simulink library "ardupilot_sitl_lib"  (R2018b)
settings: Solver=VariableStepAuto  StartTime=0.0  StopTime=10.0  RelTol=1e-3
libraries: dspnetwork x5, etargetslib x3, $bdroot x2, sensors_lib x2
settings Model: Creator=yannic  LastModifiedBy=yannic

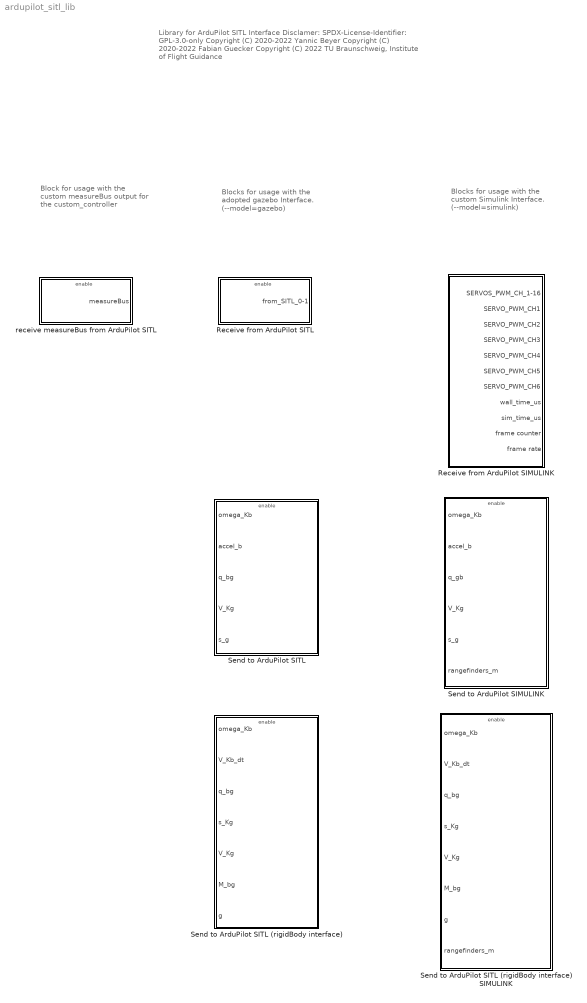
== system ardupilot_sitl_lib ==
  note: Block for usage
      | with the custom
      | measureBus output
      | for the
      | custom_controller
  note: Blocks for usage
      | with the custom
      | Simulink Interface.
      |
      | (--model=simulink)
  note: Blocks for usage
      | with the adopted
      | gazebo Interface.
      |
      | (--model=gazebo)
  note: Library for ArduPilot SITL Interface
      |
      | Disclamer:
      | SPDX-License-Identifier: GPL-3.0-only
      |
      | Copyright (C) 2020-2022 Yannic Beyer
      | Copyright (C) 2020-2022 Fabian Guecker
      | Copyright (C) 2022 TU Braunschweig, Institute of Flight Guidance
  Receive from ArduPilot SIMULINK : Subsystem  mask{IP='127.0.0.1', Port=9002, sample_time=1/400, blocking_time=1}
      mask prompts: sample_time "Sample time"; blocking_time "Blocking time (wait for signal), in s"
  Receive from ArduPilot SITL : Subsystem  mask{idx=[3,1,4,2], IP='127.0.0.1', Port=9002, sample_time=1/400, blocking_time=inf}
      mask prompts: idx "Pick channel indices"; sample_time "Sample time"; blocking_time "Blocking time (wait for signal), in s"
  Send to ArduPilot SIMULINK : Subsystem  mask{IP='127.0.0.1', Port=9003, sample_time=1/400}
      mask prompts: sample_time "Sample time"
      mask DialogControl DescGroupVar Prompt: Send to ArduPilot SITL
      mask DialogControl DescTextVar Prompt: Use rigidBody or sensor data as inputs.
      mask DialogControl Control2 Prompt: The input accel_b is the acceleration measured by an IMU in body frame.
  Send to ArduPilot SITL : Subsystem  mask{IP='127.0.0.1', Port=9003, sample_time=1/400}
      mask prompts: sample_time "Sample time"
      mask DialogControl DescGroupVar Prompt: Send to ArduPilot SITL
      mask DialogControl DescTextVar Prompt: Use rigidBody or sensor data as inputs.
      mask DialogControl Control2 Prompt: The input accel_b is the acceleration measured by an IMU in body frame.
  Send to ArduPilot SITL (rigidBody interface) : Subsystem  mask{IP='127.0.0.1', Port=9003, sample_time=1/400}
      mask prompts: sample_time "Sample time"
      mask DialogControl DescGroupVar Prompt: Send to ArduPilot SITL (rigidBody interface)
      mask DialogControl DescTextVar Prompt: Simply connect rigidBody outputs
  Send to ArduPilot SITL (rigidBody interface) SIMULINK : Subsystem  mask{IP='127.0.0.1', Port=9003, sample_time=1/400}
      mask prompts: sample_time "Sample time"
      mask DialogControl DescGroupVar Prompt: Send to ArduPilot SITL (rigidBody interface)
      mask DialogControl DescTextVar Prompt: Simply connect rigidBody outputs
  receive measureBus from ArduPilot SITL : Subsystem  mask{IP='127.0.0.1', Port=9004, sample_time=1/400, blocking_time=0.001}
      mask prompts: sample_time "Sample time"; blocking_time "Blocking time(wait for signal), in s"
      mask init:
      | num_signals = 40;
      mask DialogControl DescGroupVar Prompt: Receive measureBus from ArduPilot SITL
      mask DialogControl DescTextVar Prompt: This block can be used for debugging of the ArduPilot interface.
      mask DialogControl Control2 Prompt: This block only receives the signals if you uncomment line 3 of mode.h in your ArduPilot fork.

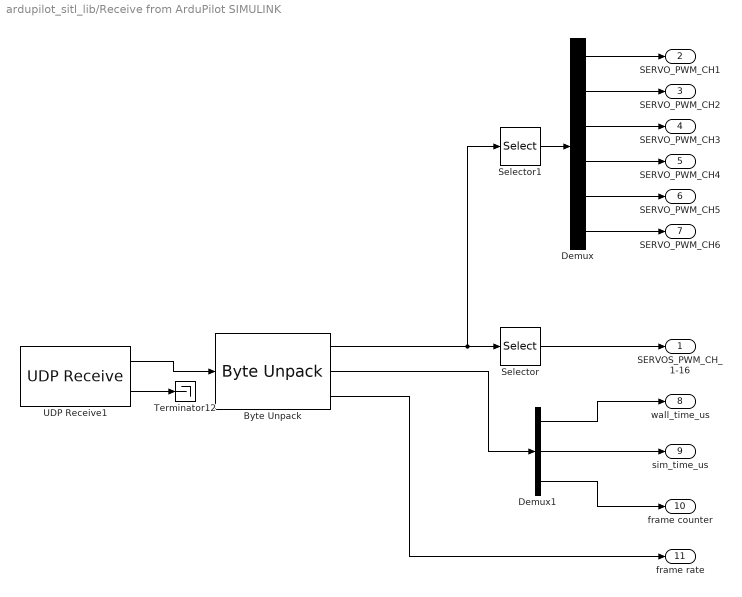
== system ardupilot_sitl_lib/Receive from ArduPilot SIMULINK ==
  Byte Unpack : etargetslib/Byte Unpack  dimensions={[16],[3],[1]}  datatypes={'double','uint32','uint16'}  byteAlign=1
      settings: SourceProductName=/root/.matlab/R2018b/slblocks_master.db is not a database. (file is encrypted or is not a database)
  Demux : Demux  Outputs=6
  Demux1 : Demux  Outputs=3
  Selector : Selector  InputPortWidth=16  IndexOptions=Index vector (dialog)  Indices=[1:16]  OutputSizes=1
  Selector1 : Selector  InputPortWidth=16  IndexOptions=Index vector (dialog)  Indices=[1:6]  OutputSizes=1
  Terminator12 : Terminator
  UDP Receive1 : dspnetwork/UDP Receive  localURL='0.0.0.0'  localPort=Port  remoteURL=IP  remotePort=-1  recvBufferSize=142  dims=142  signalDatatype=uint8  isVarSize=off  showBlockingTime=on  blockingTime=blocking_time  sampletime=sample_time  blockPlatform=HOST
      settings: SourceProductName=DSP System Toolbox  SourceProductBaseCode=DS
  SERVOS_PWM_CH_1-16 : Outport
  SERVO_PWM_CH1 : Outport  Port=2
  SERVO_PWM_CH2 : Outport  Port=3
  SERVO_PWM_CH3 : Outport  Port=4
  SERVO_PWM_CH4 : Outport  Port=5
  SERVO_PWM_CH5 : Outport  Port=6
  SERVO_PWM_CH6 : Outport  Port=7
  wall_time_us : Outport  Port=8
  sim_time_us : Outport  Port=9
  frame counter : Outport  Port=10
  frame rate : Outport  Port=11
  wires:
  UDP Receive1/1 -> Byte Unpack/1
  UDP Receive1/2 -> Terminator12/1
  Selector/1 -> SERVOS_PWM_CH_1-16/1
  Selector1/1 -> Demux/1
  Demux/1 -> SERVO_PWM_CH1/1
  Demux/2 -> SERVO_PWM_CH2/1
  Demux/6 -> SERVO_PWM_CH6/1
  Demux/5 -> SERVO_PWM_CH5/1
  Demux/4 -> SERVO_PWM_CH4/1
  Demux/3 -> SERVO_PWM_CH3/1
  Byte Unpack/2 -> Demux1/1
  Demux1/1 -> wall_time_us/1
  Demux1/2 -> sim_time_us/1
  Byte Unpack/1 -> Selector1/1, Selector/1
  Demux1/3 -> frame counter/1
  Byte Unpack/3 -> frame rate/1

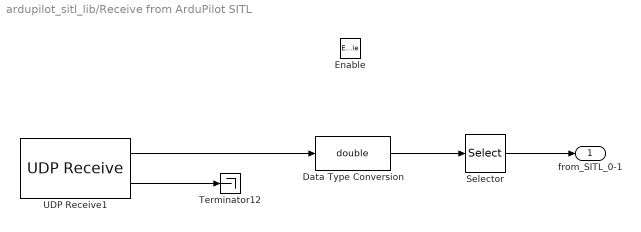
== system ardupilot_sitl_lib/Receive from ArduPilot SITL ==
  Enable : EnablePort
  Data Type Conversion : DataTypeConversion  OutDataTypeStr=double
  Selector : Selector  InputPortWidth=16  IndexOptions=Index vector (dialog)  Indices=idx  OutputSizes=1
  Terminator12 : Terminator
  UDP Receive1 : dspnetwork/UDP Receive  localURL='0.0.0.0'  localPort=Port  remoteURL=IP  remotePort=-1  recvBufferSize=64  dims=16  signalDatatype=single  isVarSize=off  showBlockingTime=on  blockingTime=blocking_time  sampletime=sample_time  blockPlatform=HOST
      settings: SourceProductName=DSP System Toolbox  SourceProductBaseCode=DS
  from_SITL_0-1 : Outport
  wires:
  UDP Receive1/1 -> Data Type Conversion/1
  UDP Receive1/2 -> Terminator12/1
  Data Type Conversion/1 -> Selector/1
  Selector/1 -> from_SITL_0-1/1

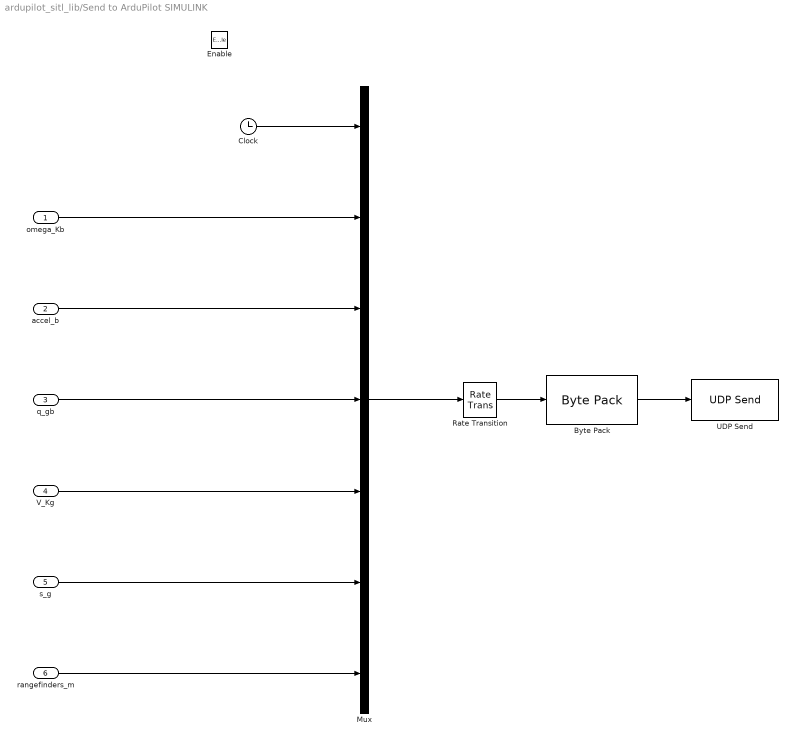
== system ardupilot_sitl_lib/Send to ArduPilot SIMULINK ==
  omega_Kb : Inport  OutDataTypeStr=double  PortDimensions=[3]
  accel_b : Inport  Port=2  OutDataTypeStr=double  PortDimensions=[3]
  q_gb : Inport  Port=3  OutDataTypeStr=double  PortDimensions=[4]
  V_Kg : Inport  Port=4  OutDataTypeStr=double  PortDimensions=[3]
  s_g : Inport  Port=5  OutDataTypeStr=double  PortDimensions=[3]
  rangefinders_m : Inport  Port=6  OutDataTypeStr=double  PortDimensions=[6]
  Enable : EnablePort
  Byte Pack : etargetslib/Byte Pack  datatypes={'double'}  byteAlign=1
      settings: SourceProductName=/root/.matlab/R2018b/slblocks_master.db is not a database. (file is encrypted or is not a database)
  Clock : Clock
  Mux : Mux  Inputs=7
  Rate Transition : RateTransition  OutPortSampleTime=sample_time
  UDP Send : dspnetwork/UDP Send  remoteURL=IP  remotePort=Port  localURL='0.0.0.0'  localPortSource=Automatically determine  localPort=-1  sampletime=-1  blockPlatform=[]  separateLengthPort=0
      settings: SourceProductName=DSP System Toolbox  SourceProductBaseCode=DS
  wires:
  q_gb/1 -> Mux/4
  omega_Kb/1 -> Mux/2
  Clock/1 -> Mux/1
  accel_b/1 -> Mux/3
  Mux/1 -> Rate Transition/1
  s_g/1 -> Mux/6
  V_Kg/1 -> Mux/5
  Rate Transition/1 -> Byte Pack/1
  Byte Pack/1 -> UDP Send/1
  rangefinders_m/1 -> Mux/7

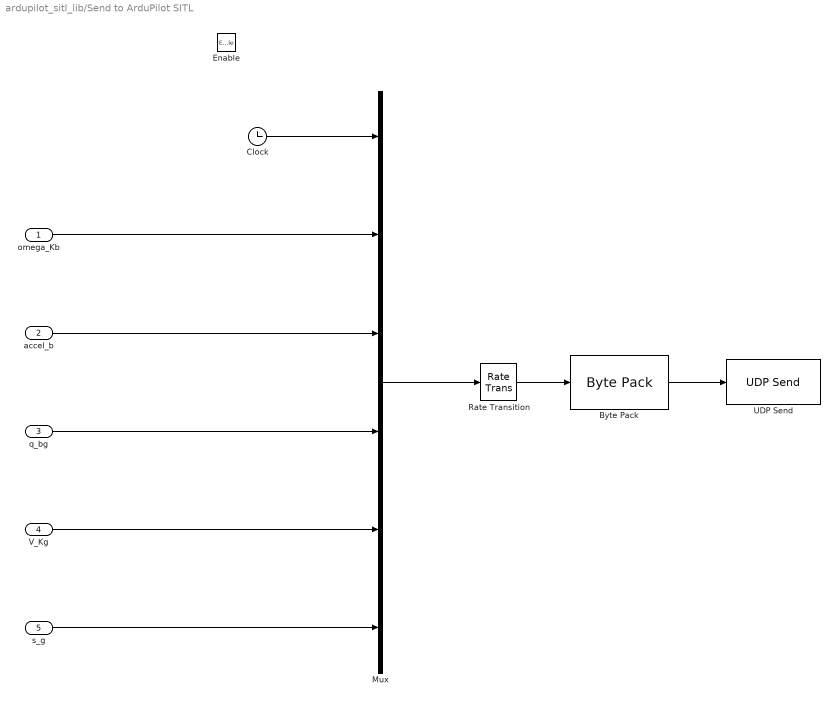
== system ardupilot_sitl_lib/Send to ArduPilot SITL ==
  omega_Kb : Inport
  accel_b : Inport  Port=2
  q_bg : Inport  Port=3
  V_Kg : Inport  Port=4
  s_g : Inport  Port=5
  Enable : EnablePort
  Byte Pack : etargetslib/Byte Pack  datatypes={'double'}  byteAlign=1
      settings: SourceProductName=/root/.matlab/R2018b/slblocks_master.db is not a database. (file is encrypted or is not a database)
  Clock : Clock
  Mux : Mux  Inputs=6
  Rate Transition : RateTransition  OutPortSampleTime=sample_time
  UDP Send : dspnetwork/UDP Send  remoteURL=IP  remotePort=Port  localURL='0.0.0.0'  localPortSource=Automatically determine  localPort=-1  sampletime=-1  blockPlatform=[]  separateLengthPort=0
      settings: SourceProductName=DSP System Toolbox  SourceProductBaseCode=DS
  wires:
  Byte Pack/1 -> UDP Send/1
  Rate Transition/1 -> Byte Pack/1
  V_Kg/1 -> Mux/5
  s_g/1 -> Mux/6
  Mux/1 -> Rate Transition/1
  accel_b/1 -> Mux/3
  Clock/1 -> Mux/1
  omega_Kb/1 -> Mux/2
  q_bg/1 -> Mux/4

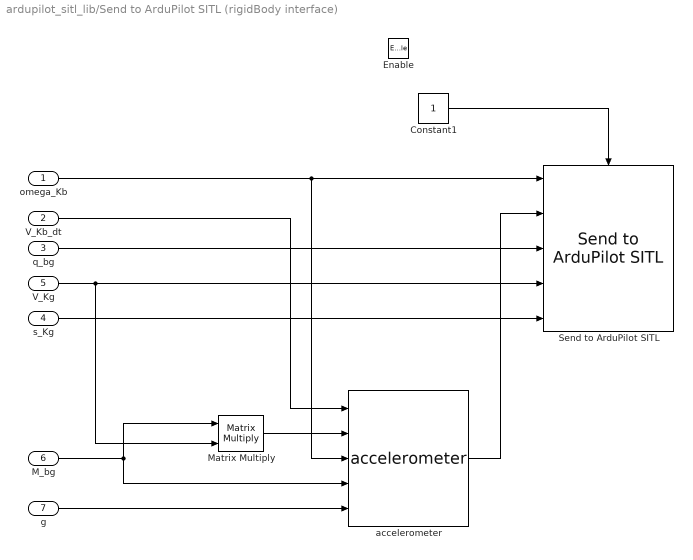
== system ardupilot_sitl_lib/Send to ArduPilot SITL (rigidBody interface) ==
  omega_Kb : Inport
  V_Kb_dt : Inport  Port=2
  q_bg : Inport  Port=3
  s_Kg : Inport  Port=4
  V_Kg : Inport  Port=5
  M_bg : Inport  Port=6
  g : Inport  Port=7
  Enable : EnablePort
  Constant1 : Constant
  Matrix Multiply : Product  Multiplication=Matrix(*)
  Send to ArduPilot SITL : $bdroot/Send to ArduPilot SITL  IP=IP  Port=Port  sample_time=sample_time
  accelerometer : sensors_lib/accelerometer  SystemSampleTime=-1
      settings: SourceProductName=LADAC
  wires:
  V_Kg/1 -> Matrix Multiply/2, Send to ArduPilot SITL/4
  q_bg/1 -> Send to ArduPilot SITL/3
  V_Kb_dt/1 -> accelerometer/1
  omega_Kb/1 -> accelerometer/3, Send to ArduPilot SITL/1
  s_Kg/1 -> Send to ArduPilot SITL/5
  M_bg/1 -> Matrix Multiply/1, accelerometer/4
  g/1 -> accelerometer/5
  accelerometer/1 -> Send to ArduPilot SITL/2
  Constant1/1 -> Send to ArduPilot SITL/Enable
  Matrix Multiply/1 -> accelerometer/2

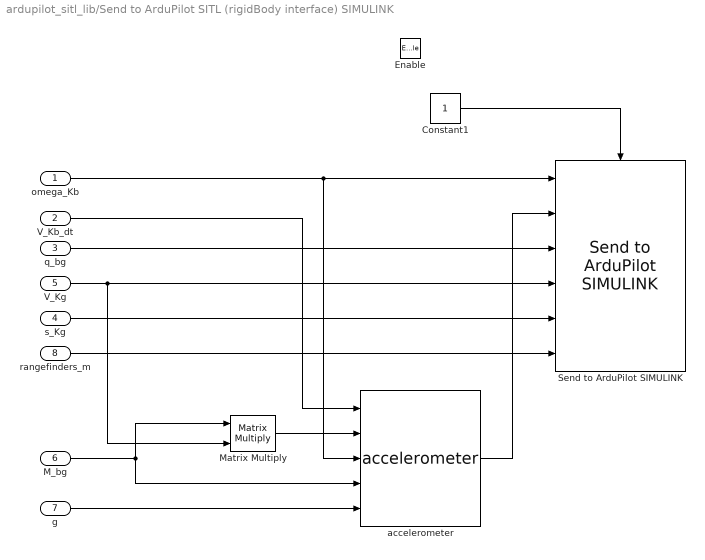
== system ardupilot_sitl_lib/Send to ArduPilot SITL (rigidBody interface) SIMULINK ==
  omega_Kb : Inport
  V_Kb_dt : Inport  Port=2
  q_bg : Inport  Port=3
  s_Kg : Inport  Port=4
  V_Kg : Inport  Port=5
  M_bg : Inport  Port=6
  g : Inport  Port=7
  rangefinders_m : Inport  Port=8
  Enable : EnablePort
  Constant1 : Constant
  Matrix Multiply : Product  Multiplication=Matrix(*)
  Send to ArduPilot SIMULINK : $bdroot/Send to ArduPilot SIMULINK  IP=IP  Port=Port  sample_time=sample_time
  accelerometer : sensors_lib/accelerometer  SystemSampleTime=-1
      settings: SourceProductName=LADAC
  wires:
  Matrix Multiply/1 -> accelerometer/2
  Constant1/1 -> Send to ArduPilot SIMULINK/Enable
  accelerometer/1 -> Send to ArduPilot SIMULINK/2
  g/1 -> accelerometer/5
  M_bg/1 -> accelerometer/4, Matrix Multiply/1
  s_Kg/1 -> Send to ArduPilot SIMULINK/5
  omega_Kb/1 -> Send to ArduPilot SIMULINK/1, accelerometer/3
  V_Kb_dt/1 -> accelerometer/1
  q_bg/1 -> Send to ArduPilot SIMULINK/3
  V_Kg/1 -> Send to ArduPilot SIMULINK/4, Matrix Multiply/2
  rangefinders_m/1 -> Send to ArduPilot SIMULINK/6

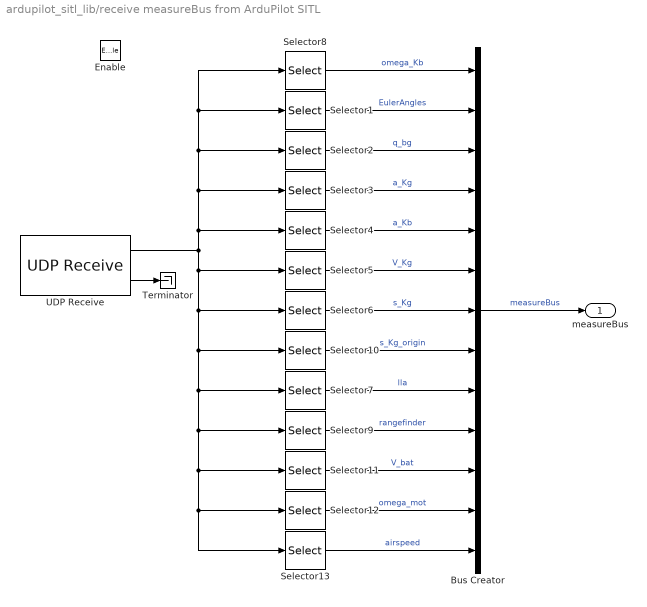
== system ardupilot_sitl_lib/receive measureBus from ArduPilot SITL ==
  Enable : EnablePort
  Bus Creator : BusCreator  Inputs=13
  Selector1 : Selector  InputPortWidth=num_signals  IndexOptions=Index vector (dialog)  Indices=4:6  OutputSizes=1
  Selector10 : Selector  InputPortWidth=num_signals  IndexOptions=Index vector (dialog)  Indices=23:25  OutputSizes=1
  Selector11 : Selector  InputPortWidth=num_signals  IndexOptions=Index vector (dialog)  Indices=35  OutputSizes=1
  Selector12 : Selector  InputPortWidth=num_signals  IndexOptions=Index vector (dialog)  Indices=36:39  OutputSizes=1
  Selector13 : Selector  InputPortWidth=num_signals  IndexOptions=Index vector (dialog)  Indices=40  OutputSizes=1
  Selector2 : Selector  InputPortWidth=num_signals  IndexOptions=Index vector (dialog)  Indices=7:10  OutputSizes=1
  Selector3 : Selector  InputPortWidth=num_signals  IndexOptions=Index vector (dialog)  Indices=11:13  OutputSizes=1
  Selector4 : Selector  InputPortWidth=num_signals  IndexOptions=Index vector (dialog)  Indices=14:16  OutputSizes=1
  Selector5 : Selector  InputPortWidth=num_signals  IndexOptions=Index vector (dialog)  Indices=17:19  OutputSizes=1
  Selector6 : Selector  InputPortWidth=num_signals  IndexOptions=Index vector (dialog)  Indices=20:22  OutputSizes=1
  Selector7 : Selector  InputPortWidth=num_signals  IndexOptions=Index vector (dialog)  Indices=26:28  OutputSizes=1
  Selector8 : Selector  InputPortWidth=num_signals  IndexOptions=Index vector (dialog)  Indices=[1,2,3]  OutputSizes=1
  Selector9 : Selector  InputPortWidth=num_signals  IndexOptions=Index vector (dialog)  Indices=29:34  OutputSizes=1
  Terminator : Terminator
  UDP Receive : dspnetwork/UDP Receive  localURL='0.0.0.0'  localPort=Port  remoteURL=IP  remotePort=-1  recvBufferSize=num_signals*4  dims=num_signals  signalDatatype=single  isVarSize=off  showBlockingTime=on  blockingTime=blocking_time  sampletime=sample_time  blockPlatform=HOST
      settings: SourceProductName=DSP System Toolbox  SourceProductBaseCode=DS
  measureBus : Outport
  wires:
  Selector4/1 -> Bus Creator/5  "a_Kb"
  Selector5/1 -> Bus Creator/6  "V_Kg"
  Selector1/1 -> Bus Creator/2  "EulerAngles"
  UDP Receive/2 -> Terminator/1
  Bus Creator/1 -> measureBus/1  "measureBus"
  Selector2/1 -> Bus Creator/3  "q_bg"
  Selector7/1 -> Bus Creator/9  "lla"
  Selector3/1 -> Bus Creator/4  "a_Kg"
  UDP Receive/1 -> Selector5/1, Selector6/1, Selector10/1, Selector13/1, Selector12/1, Selector11/1, Selector9/1, Selector7/1, Selector3/1, Selector2/1, Selector1/1, Selector8/1, Selector4/1
  Selector6/1 -> Bus Creator/7  "s_Kg"
  Selector8/1 -> Bus Creator/1  "omega_Kb"
  Selector9/1 -> Bus Creator/10  "rangefinder"
  Selector10/1 -> Bus Creator/8  "s_Kg_origin"
  Selector11/1 -> Bus Creator/11  "V_bat"
  Selector12/1 -> Bus Creator/12  "omega_mot"
  Selector13/1 -> Bus Creator/13  "airspeed"
